simulink model "ASM_Traffic_new"  (R2024a)
settings: Solver=ode1  StartTime=SIM.tstart.v  StopTime=SIM.tend.v  FixedStep=SIM.StepSize.v  RelTol=1e-3
PostLoadFcn:
  | if any(exist('dsrtsu_mdlpostloadfcn', 'file') ~= 0), dsrtsu_mdlpostloadfcn('Execute', bdroot); end
  | try, asm_mdl_postloadfcn(bdroot, 'UpdateModel', 3600); catch, disp(lasterr); end,
InitFcn:
  | , if any(exist('rtifpga_mdlclblib', 'file') ~= 0), rtifpga_mdlclblib('Init', bdroot); end,
  | , if any(exist('dsmpb_private', 'file') ~= 0), dsmpb_private('dsmpb_mdlclblib', 'Init', bdroot); end,
undefined symbols (not defined in the file): _to_, a0b2, ASM_BrakeHydraulics_DemoSystems, ASM_VehicleDynamics_DemoSystems, b98103fe8ad365046cd0, BrakeCircuit, CPT, Crankshaft, DiscIntNeverNeededParam, dsmsi, FinalDriveAssembly, MDL, ModeSignals, Pos_BrakePedal_Maneuver, rad, RefSignals, s_to_rpm, SIM, SoftECU, Suspension, Tire, Transmission
libraries: ASM_Traffic_lib x135, simulink x100, ASM_Utils_lib x77, ASM_VehicleDynamics_lib x70, ASM_Environment_lib x22, dsmpblib x20, dsmsilib x15, MDLD_Utils_lib x10, ASM_BrakeHydraulics_lib x3
(part 23 of 63)

== system ASM_Traffic_new/Environment/GroundTruth/PlantModel/HostVehicle_Data_Access ==
  OSI_HV_Data : Inport
  Enable_HostVehicle_Data_Access[0Off|1On] : Constant
  HostVehicle_Data_Access : Subsystem
  Terminator{,1..23} (24 alike) : Terminator
  wires:
  HostVehicle_Data_Access/5(HV_Position_BB[x;y;z][m]) -> Terminator4/1
  HostVehicle_Data_Access/6(HV_Velocity_BB[x;y;z][m|s]) -> Terminator5/1
  HostVehicle_Data_Access/3(HV_ID[]) -> Terminator2/1
  HostVehicle_Data_Access/4(HV_Pos_BrakePedal[0_1]) -> Terminator3/1
  HostVehicle_Data_Access/2(Time_Stamp_Nanos[ns]) -> Terminator1/1
  Enable_HostVehicle_Data_Access[0Off|1On]/1 -> HostVehicle_Data_Access/1(Enable[0Off|1On])
  OSI_HV_Data/1 -> HostVehicle_Data_Access/2(OSI_HV_Data)
  HostVehicle_Data_Access/1(Time_Stamp_Seconds[s]) -> Terminator/1
  HostVehicle_Data_Access/7(HV_Acceleration_BB[x;y;z][m|s2]) -> Terminator6/1
  HostVehicle_Data_Access/8(HV_Orientation_BB[x;y;z][rad]) -> Terminator7/1
  HostVehicle_Data_Access/9(HV_Current_Curvature[1|m]) -> Terminator8/1
  HostVehicle_Data_Access/10(HV_Steering_Angle[rad]) -> Terminator9/1
  HostVehicle_Data_Access/11(HV_Steering_Angle_dt[rad|s]) -> Terminator10/1
  HostVehicle_Data_Access/12(HV_Steering_Torque[Nm]) -> Terminator11/1
  HostVehicle_Data_Access/13(HV_Pos_AccPedal[0_1]) -> Terminator12/1
  HostVehicle_Data_Access/14(HV_Pos_ClutchPedal[0_1]) -> Terminator13/1
  HostVehicle_Data_Access/15(HV_Gear[]) -> Terminator14/1
  HostVehicle_Data_Access/16(HV_Type_Engine[]) -> Terminator15/1
  HostVehicle_Data_Access/17(HV_n_Engine[rpm]) -> Terminator16/1
  HostVehicle_Data_Access/18(HV_Trq_Engine[Nm]) -> Terminator17/1
  HostVehicle_Data_Access/19(HV_Vehicle_Weight[kg]) -> Terminator18/1
  HostVehicle_Data_Access/20(HV_Vehicle_Operating_State[]) -> Terminator19/1
  HostVehicle_Data_Access/21(HV_WheelData_Axle_Idx[]) -> Terminator20/1
  HostVehicle_Data_Access/22(HV_WheelData_Wheel_Idx[]) -> Terminator21/1
  HostVehicle_Data_Access/23(HV_WheelData_Wheel_Speed[rad|s]) -> Terminator22/1
  HostVehicle_Data_Access/24(HV_WheelData_Wheel_Slip[]) -> Terminator23/1

== system ASM_Traffic_new/Environment/GroundTruth/PlantModel/ObjectDataStreams ==
  In : Inport
  Bus Selector14 : BusSelector  OutputSignals=DataStream_1[].DataStream_1[],DataStream_2[].DataStream_2[],DataStream_3[].DataStream_3[],DataStream_4[].DataStream_4[],DataStream_5[].DataStream_5[],DataStream_6[].DataStream_6[],DataStream_7[].DataStream_7[],DataStream_8[].DataStream_8[]
  Mux : Mux  Inputs=8
  Objects_DataStreams[] : Outport  VectorParamsAs1DForOutWhenUnconnected=off
  wires:
  Mux/1 -> Objects_DataStreams[]/1
  Bus Selector14/7 -> Mux/7  "<DataStream_7[]>"
  Bus Selector14/8 -> Mux/8  "<DataStream_8[]>"
  Bus Selector14/3 -> Mux/3  "<DataStream_3[]>"
  Bus Selector14/6 -> Mux/6  "<DataStream_6[]>"
  Bus Selector14/4 -> Mux/4  "<DataStream_4[]>"
  Bus Selector14/1 -> Mux/1  "<DataStream_1[]>"
  Bus Selector14/5 -> Mux/5  "<DataStream_5[]>"
  In/1 -> Bus Selector14/1
  Bus Selector14/2 -> Mux/2  "<DataStream_2[]>"

== system ASM_Traffic_new/Environment/GroundTruth/PlantModel/Running_Maneuver ==
  ManeuverState[] : Inport
  Brake : RelationalOperator  Operator===  OutDataTypeStr=boolean  InputSameDT=off
  Constant : Constant  Value=3
  Constant1 : Constant  Value=4
  Data Type Conversion : DataTypeConversion  OutDataTypeStr=double  SaturateOnIntegerOverflow=off  RndMeth=Floor
  Logical Operator : Logic  Operator=OR  AllPortsSameDT=off  OutDataTypeStr=boolean
  Run : RelationalOperator  Operator===  OutDataTypeStr=boolean  InputSameDT=off
  EnableRun[0Off|1On] : Outport  VectorParamsAs1DForOutWhenUnconnected=off
  wires:
  Run/1 -> Logical Operator/1
  ManeuverState[]/1 -> Brake/1, Run/1
  Constant1/1 -> Brake/2
  Logical Operator/1 -> Data Type Conversion/1
  Constant/1 -> Run/2
  Brake/1 -> Logical Operator/2
  Data Type Conversion/1 -> EnableRun[0Off|1On]/1

== system ASM_Traffic_new/Environment/GroundTruth/PlantModel/TrafficLight_Counter ==
  In : Inport
  Bus Selector14 : BusSelector  OutputSignals=TrafficLight_Counter_1[].TrafficLight_Counter_1[],TrafficLight_Counter_2.TrafficLight_Counter_2[],TrafficLight_Counter_3.TrafficLight_Counter_3[],TrafficLight_Counter_4[].TrafficLight_Counter_4[]
  Mux2 : Mux
  TrafficLight_Counter[] : Outport  VectorParamsAs1DForOutWhenUnconnected=off
  wires:
  Bus Selector14/1 -> Mux2/1  "<TrafficLight_Counter_1[]>"
  In/1 -> Bus Selector14/1
  Bus Selector14/3 -> Mux2/3  "<TrafficLight_Counter_3[]>"
  Bus Selector14/2 -> Mux2/2  "<TrafficLight_Counter_2[]>"
  Bus Selector14/4 -> Mux2/4  "<TrafficLight_Counter_4[]>"
  Mux2/1 -> TrafficLight_Counter[]/1

== system ASM_Traffic_new/Environment/GroundTruth/PlantModel/VehicleBasics ==
  In : Inport
  OSIGroundTruth : Inport  Port=2
  Bus Selector : BusSelector  OutputSignals=Interface_In.ExternalModel.m_TotalVehicle[kg],Interface_In.ExternalModel.State_StartButton[-2|-1|0|1|2|3]
  Bus Selector1 : BusSelector  OutputSignals=HostVehicle_Data_VehicleBasics[].Mode_OperatingState[1Stim|2Int],HostVehicle_Data_VehicleBasics[].Stim_OperatingState[]
  Multiport Switch : MultiPortSwitch  Inputs=2  SaturateOnIntegerOverflow=off  InputSameDT=off
  StartButton_Mapping : Subsystem
  m_TotalVehicle[kg] : Outport  VectorParamsAs1DForOutWhenUnconnected=off
  OperatingState[] : Outport  Port=2  VectorParamsAs1DForOutWhenUnconnected=off
  wires:
  Multiport Switch/1 -> OperatingState[]/1  "OperatingState[]"
  Bus Selector1/2 -> Multiport Switch/2  "<Stim_OperatingState[]>"
  Bus Selector1/1 -> Multiport Switch/1  "<Mode_OperatingState[1Stim|2Int]>"
  OSIGroundTruth/1 -> Bus Selector1/1
  In/1 -> Bus Selector/1
  Bus Selector/1 -> m_TotalVehicle[kg]/1  "<m_TotalVehicle[kg]>"
  Bus Selector/2 -> StartButton_Mapping/1(State_StartButton[-2|-1|0|1|2|3])  "<State_StartButton[-2|-1|0|1|2|3]>"
  StartButton_Mapping/1(OperatingState[]) -> Multiport Switch/3

== system ASM_Traffic_new/Environment/GroundTruth/PlantModel/VehicleBrakeSystem ==
  In : Inport
  Bus Selector25 : BusSelector  OutputSignals=Interface_In.ExternalModel.Pos_BrakePedal[%]
  Gain : Gain  Gain=1/100
  Pos_BrakePedal[0_1] : Outport
  wires:
  Bus Selector25/1 -> Gain/1  "<Pos_BrakePedal[%]>"
  In/1 -> Bus Selector25/1
  Gain/1 -> Pos_BrakePedal[0_1]/1

== system ASM_Traffic_new/Environment/GroundTruth/PlantModel/VehicleLocalization ==
  In : Inport
  Bus Selector : BusSelector  OutputSignals=Longitude[deg],Latitude[deg]
  Bus Selector10 : BusSelector  OutputSignals=Maneuver.Plant.ManeuverScheduler.Parameters.Object_Type_ID[]
  Bus Selector2 : BusSelector  OutputSignals=Interface_In.ExternalModel.Pos_Vehicle_CoorSys_E[x;y;z][m]
  Bus Selector22 : BusSelector  OutputSignals=Road.Plant.UserSignals_Customized
  Bus Selector3 : BusSelector  OutputSignals=Object_Properties_Box.PosVec_x_CenterPnt_Object[m],Object_Properties_Box.PosVec_y_CenterPnt_Object[m],Object_Properties_Box.PosVec_z_CenterPnt_Object[m]
  Bus Selector4 : BusSelector  OutputSignals=Interface_In.ExternalModel.Angle_Vehicle_CoorSys_E[x;y;z][deg]
  Bus Selector5 : BusSelector  OutputSignals=Traffic.Plant.ObjectParameters.TrafficObjects.TrafficObject_Type_Data[]
  COORDINATE_TRANSFORMATION_B_TO_A : ASM_Utils_lib/MatrixOperations/COORDINATE_TRANSFORMATION_B_TO_A  ASMLibrary2Check=ASM_Traffic_lib
  ChangeLabel : Subsystem
      mask Display: disp('')
  Demux : Demux  Outputs=3
  Demux1 : Demux  Outputs=3
  GPS_POSITION : ASM_Environment_lib/Environment/Road/GPS_POSITION  Tag=ASM_SUBCOMPONENT  ASMProperties=struct('Name','GPS_POSITION','Version','3.0','Library','ASM_Environment_lib')  ASMInstanceName=GPS_Position  ASMInstanceID=2
      settings: AttributesFormatString=Instance Name: %<ASMInstanceName>\nInstance ID: %<ASMInstanceID>
  Mux : Mux  Inputs=3
  OBJECT_PROPERTIES_BOX : ASM_Traffic_lib/Objects/OBJECT_PROPERTIES_BOX  ASMProperties=struct('Name','OBJECT_PROPERTIES_BOX','Version','2.0','Library','ASM_Traffic_lib')  ASMInstanceName=object_properties_box  ASMInstanceID=1
  Terminator : Terminator
  Terminator1 : Terminator
  Pos_Veh_BoundingBox_GPS[Long;Lat;Alt][deg;deg;m] : Outport
  wires:
  Bus Selector22/1 -> GPS_POSITION/1  "<UserSignals_Customized>"
  GPS_POSITION/1 -> Terminator/1
  GPS_POSITION/2 -> Bus Selector/1
  Bus Selector/1 -> Mux/1  "<Longitude[deg]>"
  Bus Selector/2 -> Mux/2  "<Latitude[deg]>"
  Mux/1 -> Pos_Veh_BoundingBox_GPS[Long;Lat;Alt][deg;deg;m]/1
  Bus Selector10/1 -> OBJECT_PROPERTIES_BOX/1  "<Object_Type_ID[]>"
  In/1 -> Bus Selector4/1, Bus Selector5/1, Bus Selector10/1, Bus Selector2/1, Bus Selector22/1
  Bus Selector5/1 -> OBJECT_PROPERTIES_BOX/2  "<TrafficObject_Type_Data[]>"
  OBJECT_PROPERTIES_BOX/1 -> Terminator1/1
  Bus Selector2/1 -> Demux/1  "<Pos_Vehicle_CoorSys_E[x;y;z][m]>"
  Demux/1 -> COORDINATE_TRANSFORMATION_B_TO_A/1
  Demux/2 -> COORDINATE_TRANSFORMATION_B_TO_A/2
  Demux/3 -> COORDINATE_TRANSFORMATION_B_TO_A/3
  Bus Selector3/2 -> COORDINATE_TRANSFORMATION_B_TO_A/5  "<PosVec_y_CenterPnt_Object[m]>"
  Bus Selector3/1 -> COORDINATE_TRANSFORMATION_B_TO_A/4  "<PosVec_x_CenterPnt_Object[m]>"
  Bus Selector3/3 -> COORDINATE_TRANSFORMATION_B_TO_A/6  "<PosVec_z_CenterPnt_Object[m]>"
  OBJECT_PROPERTIES_BOX/2 -> Bus Selector3/1
  Demux1/1 -> COORDINATE_TRANSFORMATION_B_TO_A/7
  Demux1/2 -> COORDINATE_TRANSFORMATION_B_TO_A/8
  Demux1/3 -> COORDINATE_TRANSFORMATION_B_TO_A/9
  COORDINATE_TRANSFORMATION_B_TO_A/3 -> ChangeLabel/1(In1)  "Pos_z_CoorSysE[m]"
  COORDINATE_TRANSFORMATION_B_TO_A/1 -> GPS_POSITION/2  "Pos_x_CoorSysE[m]"
  COORDINATE_TRANSFORMATION_B_TO_A/2 -> GPS_POSITION/3  "Pos_y_CoorSysE[m]"
  Bus Selector4/1 -> Demux1/1  "<Angle_Vehicle_CoorSys_E[x;y;z][deg]>"
  ChangeLabel/1(Out1) -> Mux/3  "Altitude[m]"

== system ASM_Traffic_new/Environment/GroundTruth/PlantModel/VehiclePowertrain ==
  In : Inport
  Bus Selector : BusSelector  OutputSignals=Interface_In.ExternalModel.Pos_AccPedal[%],Interface_In.ExternalModel.Pos_ClutchPedal[%],Interface_In.ExternalModel.Gear[],Interface_In.ExternalModel.n_Engine_1[rpm],Interface_In.ExternalModel.n_Engine_2[rpm],Interface_In.ExternalModel.Type_Engine_1[0Unkown|1Other|2Otto|3Diesel|4Electric],Interface_In.ExternalModel.Type_Engine_2[0Unkown|1Other|2Otto|3Diesel|4Electric],Interface_In.ExternalModel.Trq_Engine_1[Nm],Interface_In.ExternalModel.Trq_Engine_2[Nm]
  Gain : Gain  Gain=1/100
  Gain1 : Gain  Gain=1/100
  Mux : Mux  Inputs=2
  Mux1 : Mux  Inputs=2
  Mux2 : Mux  Inputs=2
  Pos_AccPedal[0_1] : Outport  VectorParamsAs1DForOutWhenUnconnected=off
  Pos_ClutchPedal[0_1] : Outport  Port=2  VectorParamsAs1DForOutWhenUnconnected=off
  Gear[] : Outport  Port=3  VectorParamsAs1DForOutWhenUnconnected=off
  n_Engine[rpm] : Outport  Port=4  VectorParamsAs1DForOutWhenUnconnected=off
  Type_Engine[0Unkown|1Other|2Otto|3Diesel|4Electric] : Outport  Port=5  VectorParamsAs1DForOutWhenUnconnected=off
  Trq_Engine[Nm] : Outport  Port=6  VectorParamsAs1DForOutWhenUnconnected=off
  wires:
  Bus Selector/3 -> Gear[]/1  "<Gear[]>"
  Bus Selector/4 -> Mux/1  "<n_Engine_1[rpm]>"
  Bus Selector/2 -> Gain1/1  "<Pos_ClutchPedal[%]>"
  In/1 -> Bus Selector/1
  Bus Selector/1 -> Gain/1  "<Pos_AccPedal[%]>"
  Mux/1 -> n_Engine[rpm]/1
  Bus Selector/5 -> Mux/2  "<n_Engine_2[rpm]>"
  Bus Selector/6 -> Mux1/1  "<Type_Engine_1[0Unkown|1Other|2Otto|3Diesel|4Electric]>"
  Bus Selector/7 -> Mux1/2  "<Type_Engine_2[0Unkown|1Other|2Otto|3Diesel|4Electric]>"
  Bus Selector/8 -> Mux2/1  "<Trq_Engine_1[Nm]>"
  Bus Selector/9 -> Mux2/2  "<Trq_Engine_2[Nm]>"
  Mux1/1 -> Type_Engine[0Unkown|1Other|2Otto|3Diesel|4Electric]/1
  Mux2/1 -> Trq_Engine[Nm]/1
  Gain/1 -> Pos_AccPedal[0_1]/1
  Gain1/1 -> Pos_ClutchPedal[0_1]/1

== system ASM_Traffic_new/Environment/GroundTruth/PlantModel/VehicleSteering ==
  In : Inport
  Bus Selector24 : BusSelector  OutputSignals=Interface_In.ExternalModel.Angle_SteeringWheel_SteeringSystem[deg],Interface_In.ExternalModel.Angle_SteeringWheel_dt_SteeringSystem[deg|s],Interface_In.ExternalModel.Trq_SteeringWheel_SteeringSystem[Nm]
  UnitConversion : ASM_Utils_lib/UnitConversion/UnitConversion  Selection=deg_to_rad
  UnitConversion1 : ASM_Utils_lib/UnitConversion/UnitConversion  Selection=deg_to_rad
  Angle_SteeringWheel_SteeringSystem[rad] : Outport  VectorParamsAs1DForOutWhenUnconnected=off
  Angle_SteeringWheel_dt_SteeringSystem[rad|s] : Outport  Port=2  VectorParamsAs1DForOutWhenUnconnected=off
  Trq_SteeringWheel_SteeringSystem[Nm] : Outport  Port=3  VectorParamsAs1DForOutWhenUnconnected=off
  wires:
  In/1 -> Bus Selector24/1
  Bus Selector24/1 -> UnitConversion/1  "<Angle_SteeringWheel_SteeringSystem[deg]>"
  Bus Selector24/2 -> UnitConversion1/1  "<Angle_SteeringWheel_dt_SteeringSystem[deg|s]>"
  Bus Selector24/3 -> Trq_SteeringWheel_SteeringSystem[Nm]/1  "<Trq_SteeringWheel_SteeringSystem[Nm]>"
  UnitConversion/1 -> Angle_SteeringWheel_SteeringSystem[rad]/1
  UnitConversion1/1 -> Angle_SteeringWheel_dt_SteeringSystem[rad|s]/1

== system ASM_Traffic_new/Environment/GroundTruth/PlantModel/VehicleWheels ==
  In : Inport
  OSIGroundTruth : Inport  Port=2
  Bus Selector1 : BusSelector  OutputSignals=HostVehicle_Data_VehicleWheels[].Axle_Idx[],HostVehicle_Data_VehicleWheels[].Wheel_Idx[]
  Bus Selector37 : BusSelector  OutputSignals=Interface_In.ExternalModel.omega_Wheel[rad|s],Interface_In.ExternalModel.Slip_x_Wheel[]
  Axle_Idx[] : Outport  VectorParamsAs1DForOutWhenUnconnected=off
  Wheel_Idx[] : Outport  Port=2  VectorParamsAs1DForOutWhenUnconnected=off
  omega_Wheel[rad|s] : Outport  Port=3  VectorParamsAs1DForOutWhenUnconnected=off
  Slip_x_Wheel[] : Outport  Port=4  VectorParamsAs1DForOutWhenUnconnected=off
  wires:
  In/1 -> Bus Selector37/1
  Bus Selector37/1 -> omega_Wheel[rad|s]/1  "<omega_Wheel[rad|s]>"
  Bus Selector37/2 -> Slip_x_Wheel[]/1  "<Slip_x_Wheel[]>"
  Bus Selector1/1 -> Axle_Idx[]/1  "<Axle_Idx[]>"
  Bus Selector1/2 -> Wheel_Idx[]/1  "<Wheel_Idx[]>"
  OSIGroundTruth/1 -> Bus Selector1/1

== system ASM_Traffic_new/Environment/GroundTruth/UserInterface/ASMSignalBus_Plant ==
  In : Inport
  Terminator_1 : Terminator
  tag scope: ASMBUS_Traffic_GroundTruth=global
  wires:
  In/1 -> [ASMBUS_Traffic_GroundTruth]
  [ASMBUS_Traffic_GroundTruth] -> Terminator_1/1

== system ASM_Traffic_new/Environment/GroundTruth/UserInterface/DISP_Plant ==
  In : Inport
  Bus Selector : BusSelector  OutputSignals=Control.Interface_Mode[0Off|1ObjOnly|2ObjAndLanes]
  Bus Selector1 : BusSelector  OutputSignals=Data_Access.Num_MovObj[],Data_Access.Num_MovObj_in_GT_Area[],Data_Access.Num_StatObj[],Data_Access.Num_StatObj_in_GT_Area[],Data_Access.Num_Laneboundaries[],Data_Access.Num_Lanes[],Data_Access.Num_TrfLights[],Data_Access.Num_TrfLights_in_GT_Area[],Data_Access.Num_TrfSigns[],Data_Access.Num_TrfSigns_in_GT_Area[]
  Bus Selector2 : BusSelector  OutputSignals=Data_Access.Num_MovObj[],Data_Access.Num_MovObj_in_GT_Area[],Data_Access.Num_StatObj[],Data_Access.Num_StatObj_in_GT_Area[],Data_Access.Num_Laneboundaries[],Data_Access.Num_Lanes[],Data_Access.Num_TrfLights[],Data_Access.Num_TrfLights_in_GT_Area[],Data_Access.Num_TrfSigns[],Data_Access.Num_TrfSigns_in_GT_Area[]
  Interface_Mode : Scope
  Interface_Mode[0Off|1ObjOnly|2ObjAndLanes] : Subsystem
      mask Display: disp('')
  Interface_Mode_Disp : Display
  Lanes_Laneboundaries : Scope  NumInputPorts=2
  MovObj : Scope  NumInputPorts=2
  Num_Laneboundaries : Display
  Num_Laneboundaries[] : Subsystem
      mask Display: disp('')
  Num_Lanes : Display
  Num_Lanes[] : Subsystem
      mask Display: disp('')
  Num_MovObj : Display
  Num_MovObj[] : Subsystem
      mask Display: disp('')
  Num_MovObj_in_GT_Area : Display
  Num_MovObj_in_GT_Area[] : Subsystem
      mask Display: disp('')
  Num_StatObj : Display
  Num_StatObj[] : Subsystem
      mask Display: disp('')
  Num_StatObj_in_GT_Area : Display
  Num_StatObj_in_GT_Area[] : Subsystem
      mask Display: disp('')
  Num_TrfLights : Display
  Num_TrfLights[] : Subsystem
      mask Display: disp('')
  Num_TrfLights_in_GT_Area : Display
  Num_TrfLights_in_GT_Area[] : Subsystem
      mask Display: disp('')
  Num_TrfSigns : Display
  Num_TrfSigns[] : Subsystem
      mask Display: disp('')
  Num_TrfSigns_in_GT_Area : Display
  Num_TrfSigns_in_GT_Area[] : Subsystem
      mask Display: disp('')
  StatObj : Scope  NumInputPorts=2
  TrfLights : Scope  NumInputPorts=2
  TrfSigns : Scope  NumInputPorts=2
  wires:
  In/1 -> Bus Selector2/1, Bus Selector1/1, Bus Selector/1
  Bus Selector/1 -> Interface_Mode[0Off|1ObjOnly|2ObjAndLanes]/1(In1)  "<Interface_Mode[0Off|1ObjOnly|2ObjAndLanes]>"
  Bus Selector1/1 -> Num_MovObj[]/1(In1)  "<Num_MovObj[]>"
  Bus Selector1/2 -> Num_MovObj_in_GT_Area[]/1(In1)  "<Num_MovObj_in_GT_Area[]>"
  Bus Selector1/3 -> Num_StatObj[]/1(In1)  "<Num_StatObj[]>"
  Bus Selector1/4 -> Num_StatObj_in_GT_Area[]/1(In1)  "<Num_StatObj_in_GT_Area[]>"
  Bus Selector1/5 -> Num_Laneboundaries[]/1(In1)  "<Num_Laneboundaries[]>"
  Bus Selector1/6 -> Num_Lanes[]/1(In1)  "<Num_Lanes[]>"
  Bus Selector1/7 -> Num_TrfLights[]/1(In1)  "<Num_TrfLights[]>"
  Bus Selector1/8 -> Num_TrfLights_in_GT_Area[]/1(In1)  "<Num_TrfLights_in_GT_Area[]>"
  Bus Selector1/9 -> Num_TrfSigns[]/1(In1)  "<Num_TrfSigns[]>"
  Bus Selector1/10 -> Num_TrfSigns_in_GT_Area[]/1(In1)  "<Num_TrfSigns_in_GT_Area[]>"
  Num_MovObj[]/1(Out1) -> MovObj/1  "Num_MovObj[]"
  Num_MovObj_in_GT_Area[]/1(Out1) -> MovObj/2  "Num_MovObj_in_GT_Area[]"
  Interface_Mode[0Off|1ObjOnly|2ObjAndLanes]/1(Out1) -> Interface_Mode_Disp/1, Interface_Mode/1  "Interface_Mode[0Off|1ObjOnly|2ObjAndLanes]"
  Num_StatObj[]/1(Out1) -> StatObj/1  "Num_StatObj[]"
  Num_StatObj_in_GT_Area[]/1(Out1) -> StatObj/2  "Num_StatObj_in_GT_Area[]"
  Num_Laneboundaries[]/1(Out1) -> Lanes_Laneboundaries/1  "Num_Laneboundaries[]"
  Num_Lanes[]/1(Out1) -> Lanes_Laneboundaries/2  "Num_Lanes[]"
  Num_TrfLights[]/1(Out1) -> TrfLights/1  "Num_TrfLights[]"
  Num_TrfLights_in_GT_Area[]/1(Out1) -> TrfLights/2  "Num_TrfLights_in_GT_Area[]"
  Num_TrfSigns[]/1(Out1) -> TrfSigns/1  "Num_TrfSigns[]"
  Num_TrfSigns_in_GT_Area[]/1(Out1) -> TrfSigns/2  "Num_TrfSigns_in_GT_Area[]"
  Bus Selector2/1 -> Num_MovObj/1  "<Num_MovObj[]>"
  Bus Selector2/2 -> Num_MovObj_in_GT_Area/1  "<Num_MovObj_in_GT_Area[]>"
  Bus Selector2/3 -> Num_StatObj/1  "<Num_StatObj[]>"
  Bus Selector2/4 -> Num_StatObj_in_GT_Area/1  "<Num_StatObj_in_GT_Area[]>"
  Bus Selector2/5 -> Num_Laneboundaries/1  "<Num_Laneboundaries[]>"
  Bus Selector2/6 -> Num_Lanes/1  "<Num_Lanes[]>"
  Bus Selector2/7 -> Num_TrfLights/1  "<Num_TrfLights[]>"
  Bus Selector2/8 -> Num_TrfLights_in_GT_Area/1  "<Num_TrfLights_in_GT_Area[]>"
  Bus Selector2/9 -> Num_TrfSigns/1  "<Num_TrfSigns[]>"
  Bus Selector2/10 -> Num_TrfSigns_in_GT_Area/1  "<Num_TrfSigns_in_GT_Area[]>"

== system ASM_Traffic_new/Environment/GroundTruth/UserInterface/PAR_Plant ==
  Interface_In : Inport
  In : Inport  Port=2
  Bus Creator : BusCreator  Inputs=1
  Bus Creator1 : BusCreator  Inputs=9
  Country_Code[] : Constant  Tag=AD:ASM_Sw_SpeedLimit_Source[1Manual|2RoadScenery]
  Ego_Vehicle : Subsystem
  Enable_HostVehicle_Data[0Off|1On] : Constant  Tag=AD:ASM_Sw_SpeedLimit_Source[1Manual|2RoadScenery]
  Environmental_Conditions : Subsystem
  Fellow_Vehicles : Subsystem
  HostVehicle_Data_AutomatedDrivingFunction : Subsystem
  HostVehicle_Data_VehicleBasics : Subsystem
  HostVehicle_Data_VehicleWheels : Subsystem
  Terminator1 : Terminator
  TrafficLight_Counter : Subsystem
  Out : Outport  VectorParamsAs1DForOutWhenUnconnected=off
  wires:
  In/1 -> Terminator1/1
  Bus Creator/1 -> Out/1  "UserInterface"
  Bus Creator1/1 -> Bus Creator/1  "OSIGroundTruth"
  Enable_HostVehicle_Data[0Off|1On]/1 -> Bus Creator1/6  "Enable_HostVehicle_Data[0Off|1On]"
  HostVehicle_Data_VehicleWheels/1(HostVehicle_Data_VehicleWheels[]) -> Bus Creator1/7
  Ego_Vehicle/1(Ego_Vehicle[]) -> Bus Creator1/2
  Country_Code[]/1 -> Bus Creator1/1  "Country_Code[]"
  Fellow_Vehicles/1(Fellow_Vehicles[]) -> Bus Creator1/3
  Interface_In/1 -> HostVehicle_Data_AutomatedDrivingFunction/1(Interface_In), Fellow_Vehicles/1(Interface_In), Ego_Vehicle/1(Interface_In)
  Environmental_Conditions/1(Environmental_Conditions[]) -> Bus Creator1/4
  TrafficLight_Counter/1(TrafficLight_Counter[]) -> Bus Creator1/5
  HostVehicle_Data_AutomatedDrivingFunction/1(HostVehicle_Data_AutomatedDrivingFunction[]) -> Bus Creator1/9
  HostVehicle_Data_VehicleBasics/1(HostVehicle_Data_VehicleBasics[]) -> Bus Creator1/8

== system ASM_Traffic_new/Environment/Interface_In/ModelSignals/ACC_State[1OFF|2Standby|3ON]_ ==
  In1 : Inport
  DummyGain : Gain  SaturateOnIntegerOverflow=on  OutDataTypeStr=Inherit: Same as input  ParamDataTypeStr=Inherit: Same as input
  Out1 : Outport  VectorParamsAs1DForOutWhenUnconnected=off
  wires:
  DummyGain/1 -> Out1/1
  In1/1 -> DummyGain/1

== system ASM_Traffic_new/Environment/Interface_In/ModelSignals/AEB[0|1]_ ==
  In1 : Inport
  Gain : Gain  SaturateOnIntegerOverflow=on  OutDataTypeStr=Inherit: Same as input  ParamDataTypeStr=Inherit: Same as input
  Out1 : Outport  VectorParamsAs1DForOutWhenUnconnected=off
  wires:
  Gain/1 -> Out1/1
  In1/1 -> Gain/1

== system ASM_Traffic_new/Environment/Interface_In/ModelSignals/Active_CP_VehDyn_Trailer[]_ ==
  In1 : Inport
  Gain : Gain  SaturateOnIntegerOverflow=on  OutDataTypeStr=Inherit: Same as input  ParamDataTypeStr=Inherit: Same as input
  Out1 : Outport  VectorParamsAs1DForOutWhenUnconnected=off
  wires:
  In1/1 -> Gain/1
  Gain/1 -> Out1/1

== system ASM_Traffic_new/Environment/Interface_In/ModelSignals/Angle_SteeringWheel[deg]_ ==
  In1 : Inport
  DummyGain : Gain  SaturateOnIntegerOverflow=on  OutDataTypeStr=Inherit: Same as input  ParamDataTypeStr=Inherit: Same as input
  Out1 : Outport  VectorParamsAs1DForOutWhenUnconnected=off
  wires:
  DummyGain/1 -> Out1/1
  In1/1 -> DummyGain/1

== system ASM_Traffic_new/Environment/Interface_In/ModelSignals/Angle_SteeringWheel_SteeringSystem[deg]_ ==
  In1 : Inport
  Gain : Gain  SaturateOnIntegerOverflow=on  OutDataTypeStr=Inherit: Same as input  ParamDataTypeStr=Inherit: Same as input
  Out1 : Outport  VectorParamsAs1DForOutWhenUnconnected=off
  wires:
  Gain/1 -> Out1/1
  In1/1 -> Gain/1

== system ASM_Traffic_new/Environment/Interface_In/ModelSignals/Angle_SteeringWheel_dt_SteeringSystem[deg|s]_ ==
  In1 : Inport
  Gain : Gain  SaturateOnIntegerOverflow=on  OutDataTypeStr=Inherit: Same as input  ParamDataTypeStr=Inherit: Same as input
  Out1 : Outport  VectorParamsAs1DForOutWhenUnconnected=off
  wires:
  Gain/1 -> Out1/1
  In1/1 -> Gain/1

== system ASM_Traffic_new/Environment/Interface_In/ModelSignals/Angle_Vehicle_CoorSys_E[x;y;z][deg]_ ==
  In1 : Inport
  Gain : Gain  SaturateOnIntegerOverflow=on  OutDataTypeStr=Inherit: Same as input  ParamDataTypeStr=Inherit: Same as input
  Out1 : Outport  VectorParamsAs1DForOutWhenUnconnected=off
  wires:
  Gain/1 -> Out1/1
  In1/1 -> Gain/1

== system ASM_Traffic_new/Environment/Interface_In/ModelSignals/Coef_RollingRes[FL;FR;RL;RR][]_ ==
  In1 : Inport
  Gain : Gain  SaturateOnIntegerOverflow=on  OutDataTypeStr=Inherit: Same as input  ParamDataTypeStr=Inherit: Same as input
  Out1 : Outport  VectorParamsAs1DForOutWhenUnconnected=off
  wires:
  Gain/1 -> Out1/1
  In1/1 -> Gain/1

== system ASM_Traffic_new/Environment/Interface_In/ModelSignals/Coef_RollingRes_Mean[]_ ==
  In1 : Inport
  Gain : Gain  SaturateOnIntegerOverflow=on  OutDataTypeStr=Inherit: Same as input  ParamDataTypeStr=Inherit: Same as input
  Out1 : Outport  VectorParamsAs1DForOutWhenUnconnected=off
  wires:
  In1/1 -> Gain/1
  Gain/1 -> Out1/1

== system ASM_Traffic_new/Environment/Interface_In/ModelSignals/Const_r_unloaded_Tire_Mean[m]_ ==
  In1 : Inport
  Gain : Gain  SaturateOnIntegerOverflow=on  OutDataTypeStr=Inherit: Same as input  ParamDataTypeStr=Inherit: Same as input
  Out1 : Outport  VectorParamsAs1DForOutWhenUnconnected=off
  wires:
  In1/1 -> Gain/1
  Gain/1 -> Out1/1

== system ASM_Traffic_new/Environment/Interface_In/ModelSignals/CorneringStiffness[FL;FR;RL;RR][N]_ ==
  In1 : Inport
  Gain : Gain  SaturateOnIntegerOverflow=on  OutDataTypeStr=Inherit: Same as input  ParamDataTypeStr=Inherit: Same as input
  Out1 : Outport  VectorParamsAs1DForOutWhenUnconnected=off
  wires:
  Gain/1 -> Out1/1
  In1/1 -> Gain/1

== system ASM_Traffic_new/Environment/Interface_In/ModelSignals/Driver_Override_ACC_Active[0Off|1On]_ ==
  In1 : Inport
  DummyGain : Gain  SaturateOnIntegerOverflow=on  OutDataTypeStr=Inherit: Same as input  ParamDataTypeStr=Inherit: Same as input
  Out1 : Outport  VectorParamsAs1DForOutWhenUnconnected=off
  wires:
  DummyGain/1 -> Out1/1
  In1/1 -> DummyGain/1

== system ASM_Traffic_new/Environment/Interface_In/ModelSignals/Driver_Override_ACC_Reason[0NoOverride|1BrakePedal|2AccPedal]_ ==
  In1 : Inport
  DummyGain : Gain  SaturateOnIntegerOverflow=on  OutDataTypeStr=Inherit: Same as input  ParamDataTypeStr=Inherit: Same as input
  Out1 : Outport  VectorParamsAs1DForOutWhenUnconnected=off
  wires:
  DummyGain/1 -> Out1/1
  In1/1 -> DummyGain/1

== system ASM_Traffic_new/Environment/Interface_In/ModelSignals/FCW[0|1]_ ==
  In1 : Inport
  Gain : Gain  SaturateOnIntegerOverflow=on  OutDataTypeStr=Inherit: Same as input  ParamDataTypeStr=Inherit: Same as input
  Out1 : Outport  VectorParamsAs1DForOutWhenUnconnected=off
  wires:
  Gain/1 -> Out1/1
  In1/1 -> Gain/1

== system ASM_Traffic_new/Environment/Interface_In/ModelSignals/Gear[]_ ==
  In1 : Inport
  DummyGain : Gain  SaturateOnIntegerOverflow=on  OutDataTypeStr=Inherit: Same as input  ParamDataTypeStr=Inherit: Same as input
  Out1 : Outport  VectorParamsAs1DForOutWhenUnconnected=off
  wires:
  In1/1 -> DummyGain/1
  DummyGain/1 -> Out1/1

== system ASM_Traffic_new/Environment/Interface_In/ModelSignals/Mode_Drivetrain[1|2|3|4|5]_ ==
  In1 : Inport
  Gain : Gain  SaturateOnIntegerOverflow=on  OutDataTypeStr=Inherit: Same as input  ParamDataTypeStr=Inherit: Same as input
  Out1 : Outport  VectorParamsAs1DForOutWhenUnconnected=off
  wires:
  In1/1 -> Gain/1
  Gain/1 -> Out1/1

== system ASM_Traffic_new/Environment/Interface_In/ModelSignals/Mode_Transmission[1Manual|2Automatic]_ ==
  In1 : Inport
  Gain : Gain  SaturateOnIntegerOverflow=on  OutDataTypeStr=Inherit: Same as input  ParamDataTypeStr=Inherit: Same as input
  Out1 : Outport  VectorParamsAs1DForOutWhenUnconnected=off
  wires:
  In1/1 -> Gain/1
  Gain/1 -> Out1/1

== system ASM_Traffic_new/Environment/Interface_In/ModelSignals/Pos_AccPedal[%]_ ==
  In1 : Inport
  DummyGain : Gain  SaturateOnIntegerOverflow=on  OutDataTypeStr=Inherit: Same as input  ParamDataTypeStr=Inherit: Same as input
  Out1 : Outport  VectorParamsAs1DForOutWhenUnconnected=off
  wires:
  In1/1 -> DummyGain/1
  DummyGain/1 -> Out1/1

== system ASM_Traffic_new/Environment/Interface_In/ModelSignals/Pos_BrakePedal[%]_ ==
  In1 : Inport
  DummyGain : Gain  SaturateOnIntegerOverflow=on  OutDataTypeStr=Inherit: Same as input  ParamDataTypeStr=Inherit: Same as input
  Out1 : Outport  VectorParamsAs1DForOutWhenUnconnected=off
  wires:
  In1/1 -> DummyGain/1
  DummyGain/1 -> Out1/1

== system ASM_Traffic_new/Environment/Interface_In/ModelSignals/Pos_CP_FL2_Trailer_CoorSys_E[x;y][m]_ ==
  In1 : Inport
  Gain : Gain  SaturateOnIntegerOverflow=on  OutDataTypeStr=Inherit: Same as input  ParamDataTypeStr=Inherit: Same as input
  Out1 : Outport  VectorParamsAs1DForOutWhenUnconnected=off
  wires:
  Gain/1 -> Out1/1
  In1/1 -> Gain/1

== system ASM_Traffic_new/Environment/Interface_In/ModelSignals/Pos_CP_FL_CoorSys_E[x;y][m]_ ==
  In1 : Inport
  Gain : Gain  SaturateOnIntegerOverflow=on  OutDataTypeStr=Inherit: Same as input  ParamDataTypeStr=Inherit: Same as input
  Out1 : Outport  VectorParamsAs1DForOutWhenUnconnected=off
  wires:
  Gain/1 -> Out1/1
  In1/1 -> Gain/1

== system ASM_Traffic_new/Environment/Interface_In/ModelSignals/Pos_CP_FL_Trailer_CoorSys_E[x;y][m]_ ==
  In1 : Inport
  Gain : Gain  SaturateOnIntegerOverflow=on  OutDataTypeStr=Inherit: Same as input  ParamDataTypeStr=Inherit: Same as input
  Out1 : Outport  VectorParamsAs1DForOutWhenUnconnected=off
  wires:
  Gain/1 -> Out1/1
  In1/1 -> Gain/1

== system ASM_Traffic_new/Environment/Interface_In/ModelSignals/Pos_CP_FR2_Trailer_CoorSys_E[x;y][m]_ ==
  In1 : Inport
  Gain : Gain  SaturateOnIntegerOverflow=on  OutDataTypeStr=Inherit: Same as input  ParamDataTypeStr=Inherit: Same as input
  Out1 : Outport  VectorParamsAs1DForOutWhenUnconnected=off
  wires:
  Gain/1 -> Out1/1
  In1/1 -> Gain/1

== system ASM_Traffic_new/Environment/Interface_In/ModelSignals/Pos_CP_FR_CoorSys_E[x;y][m]_ ==
  In1 : Inport
  Gain : Gain  SaturateOnIntegerOverflow=on  OutDataTypeStr=Inherit: Same as input  ParamDataTypeStr=Inherit: Same as input
  Out1 : Outport  VectorParamsAs1DForOutWhenUnconnected=off
  wires:
  In1/1 -> Gain/1
  Gain/1 -> Out1/1

== system ASM_Traffic_new/Environment/Interface_In/ModelSignals/Pos_CP_FR_Trailer_CoorSys_E[x;y][m]_ ==
  In1 : Inport
  Gain : Gain  SaturateOnIntegerOverflow=on  OutDataTypeStr=Inherit: Same as input  ParamDataTypeStr=Inherit: Same as input
  Out1 : Outport  VectorParamsAs1DForOutWhenUnconnected=off
  wires:
  Gain/1 -> Out1/1
  In1/1 -> Gain/1

== system ASM_Traffic_new/Environment/Interface_In/ModelSignals/Pos_CP_Front_CoorSys_E[x;y][m]_ ==
  In1 : Inport
  Gain : Gain  SaturateOnIntegerOverflow=on  OutDataTypeStr=Inherit: Same as input  ParamDataTypeStr=Inherit: Same as input
  Out1 : Outport  VectorParamsAs1DForOutWhenUnconnected=off
  wires:
  In1/1 -> Gain/1
  Gain/1 -> Out1/1

== system ASM_Traffic_new/Environment/Interface_In/ModelSignals/Pos_CP_R2L2_CoorSys_E[x;y][m]_ ==
  In1 : Inport
  Gain : Gain  SaturateOnIntegerOverflow=on  OutDataTypeStr=Inherit: Same as input  ParamDataTypeStr=Inherit: Same as input
  Out1 : Outport  VectorParamsAs1DForOutWhenUnconnected=off
  wires:
  In1/1 -> Gain/1
  Gain/1 -> Out1/1

== system ASM_Traffic_new/Environment/Interface_In/ModelSignals/Pos_CP_R2L2_Trailer_CoorSys_E[x;y][m]_ ==
  In1 : Inport
  Gain : Gain  SaturateOnIntegerOverflow=on  OutDataTypeStr=Inherit: Same as input  ParamDataTypeStr=Inherit: Same as input
  Out1 : Outport  VectorParamsAs1DForOutWhenUnconnected=off
  wires:
  Gain/1 -> Out1/1
  In1/1 -> Gain/1

== system ASM_Traffic_new/Environment/Interface_In/ModelSignals/Pos_CP_R2L_CoorSys_E[x;y][m]_ ==
  In1 : Inport
  Gain : Gain  SaturateOnIntegerOverflow=on  OutDataTypeStr=Inherit: Same as input  ParamDataTypeStr=Inherit: Same as input
  Out1 : Outport  VectorParamsAs1DForOutWhenUnconnected=off
  wires:
  Gain/1 -> Out1/1
  In1/1 -> Gain/1

== system ASM_Traffic_new/Environment/Interface_In/ModelSignals/Pos_CP_R2L_Trailer_CoorSys_E[x;y][m]_ ==
  In1 : Inport
  Gain : Gain  SaturateOnIntegerOverflow=on  OutDataTypeStr=Inherit: Same as input  ParamDataTypeStr=Inherit: Same as input
  Out1 : Outport  VectorParamsAs1DForOutWhenUnconnected=off
  wires:
  Gain/1 -> Out1/1
  In1/1 -> Gain/1

== system ASM_Traffic_new/Environment/Interface_In/ModelSignals/Pos_CP_R2R2_CoorSys_E[x;y][m]_ ==
  In1 : Inport
  Gain : Gain  SaturateOnIntegerOverflow=on  OutDataTypeStr=Inherit: Same as input  ParamDataTypeStr=Inherit: Same as input
  Out1 : Outport  VectorParamsAs1DForOutWhenUnconnected=off
  wires:
  In1/1 -> Gain/1
  Gain/1 -> Out1/1

== system ASM_Traffic_new/Environment/Interface_In/ModelSignals/Pos_CP_R2R2_Trailer_CoorSys_E[x;y][m]_ ==
  In1 : Inport
  Gain : Gain  SaturateOnIntegerOverflow=on  OutDataTypeStr=Inherit: Same as input  ParamDataTypeStr=Inherit: Same as input
  Out1 : Outport  VectorParamsAs1DForOutWhenUnconnected=off
  wires:
  Gain/1 -> Out1/1
  In1/1 -> Gain/1

== system ASM_Traffic_new/Environment/Interface_In/ModelSignals/Pos_CP_R2R_CoorSys_E[x;y][m]_ ==
  In1 : Inport
  Gain : Gain  SaturateOnIntegerOverflow=on  OutDataTypeStr=Inherit: Same as input  ParamDataTypeStr=Inherit: Same as input
  Out1 : Outport  VectorParamsAs1DForOutWhenUnconnected=off
  wires:
  Gain/1 -> Out1/1
  In1/1 -> Gain/1

== system ASM_Traffic_new/Environment/Interface_In/ModelSignals/Pos_CP_R2R_Trailer_CoorSys_E[x;y][m]_ ==
  In1 : Inport
  Gain : Gain  SaturateOnIntegerOverflow=on  OutDataTypeStr=Inherit: Same as input  ParamDataTypeStr=Inherit: Same as input
  Out1 : Outport  VectorParamsAs1DForOutWhenUnconnected=off
  wires:
  Gain/1 -> Out1/1
  In1/1 -> Gain/1

== system ASM_Traffic_new/Environment/Interface_In/ModelSignals/Pos_CP_RL2_CoorSys_E[x;y][m]_ ==
  In1 : Inport
  Gain : Gain  SaturateOnIntegerOverflow=on  OutDataTypeStr=Inherit: Same as input  ParamDataTypeStr=Inherit: Same as input
  Out1 : Outport  VectorParamsAs1DForOutWhenUnconnected=off
  wires:
  In1/1 -> Gain/1
  Gain/1 -> Out1/1

== system ASM_Traffic_new/Environment/Interface_In/ModelSignals/Pos_CP_RL2_Trailer_CoorSys_E[x;y][m]_ ==
  In1 : Inport
  Gain : Gain  SaturateOnIntegerOverflow=on  OutDataTypeStr=Inherit: Same as input  ParamDataTypeStr=Inherit: Same as input
  Out1 : Outport  VectorParamsAs1DForOutWhenUnconnected=off
  wires:
  Gain/1 -> Out1/1
  In1/1 -> Gain/1

== system ASM_Traffic_new/Environment/Interface_In/ModelSignals/Pos_CP_RL_CoorSys_E[x;y][m]_ ==
  In1 : Inport
  Gain : Gain  SaturateOnIntegerOverflow=on  OutDataTypeStr=Inherit: Same as input  ParamDataTypeStr=Inherit: Same as input
  Out1 : Outport  VectorParamsAs1DForOutWhenUnconnected=off
  wires:
  Gain/1 -> Out1/1
  In1/1 -> Gain/1

== system ASM_Traffic_new/Environment/Interface_In/ModelSignals/Pos_CP_RL_Trailer_CoorSys_E[x;y][m]_ ==
  In1 : Inport
  Gain : Gain  SaturateOnIntegerOverflow=on  OutDataTypeStr=Inherit: Same as input  ParamDataTypeStr=Inherit: Same as input
  Out1 : Outport  VectorParamsAs1DForOutWhenUnconnected=off
  wires:
  Gain/1 -> Out1/1
  In1/1 -> Gain/1

== system ASM_Traffic_new/Environment/Interface_In/ModelSignals/Pos_CP_RR2_CoorSys_E[x;y][m]_ ==
  In1 : Inport
  Gain : Gain  SaturateOnIntegerOverflow=on  OutDataTypeStr=Inherit: Same as input  ParamDataTypeStr=Inherit: Same as input
  Out1 : Outport  VectorParamsAs1DForOutWhenUnconnected=off
  wires:
  In1/1 -> Gain/1
  Gain/1 -> Out1/1

== system ASM_Traffic_new/Environment/Interface_In/ModelSignals/Pos_CP_RR2_Trailer_CoorSys_E[x;y][m]_ ==
  In1 : Inport
  Gain : Gain  SaturateOnIntegerOverflow=on  OutDataTypeStr=Inherit: Same as input  ParamDataTypeStr=Inherit: Same as input
  Out1 : Outport  VectorParamsAs1DForOutWhenUnconnected=off
  wires:
  Gain/1 -> Out1/1
  In1/1 -> Gain/1

== system ASM_Traffic_new/Environment/Interface_In/ModelSignals/Pos_CP_RR_CoorSys_E[x;y][m]_ ==
  In1 : Inport
  Gain : Gain  SaturateOnIntegerOverflow=on  OutDataTypeStr=Inherit: Same as input  ParamDataTypeStr=Inherit: Same as input
  Out1 : Outport  VectorParamsAs1DForOutWhenUnconnected=off
  wires:
  Gain/1 -> Out1/1
  In1/1 -> Gain/1

== system ASM_Traffic_new/Environment/Interface_In/ModelSignals/Pos_CP_RR_Trailer_CoorSys_E[x;y][m]_ ==
  In1 : Inport
  Gain : Gain  SaturateOnIntegerOverflow=on  OutDataTypeStr=Inherit: Same as input  ParamDataTypeStr=Inherit: Same as input
  Out1 : Outport  VectorParamsAs1DForOutWhenUnconnected=off
  wires:
  Gain/1 -> Out1/1
  In1/1 -> Gain/1

== system ASM_Traffic_new/Environment/Interface_In/ModelSignals/Pos_CP_Rear_CoorSys_E[x;y][m]_ ==
  In1 : Inport
  Gain : Gain  SaturateOnIntegerOverflow=on  OutDataTypeStr=Inherit: Same as input  ParamDataTypeStr=Inherit: Same as input
  Out1 : Outport  VectorParamsAs1DForOutWhenUnconnected=off
  wires:
  Gain/1 -> Out1/1
  In1/1 -> Gain/1

== system ASM_Traffic_new/Environment/Interface_In/ModelSignals/Pos_ClutchPedal[%]_ ==
  In1 : Inport
  DummyGain : Gain  SaturateOnIntegerOverflow=on  OutDataTypeStr=Inherit: Same as input  ParamDataTypeStr=Inherit: Same as input
  Out1 : Outport  VectorParamsAs1DForOutWhenUnconnected=off
  wires:
  In1/1 -> DummyGain/1
  DummyGain/1 -> Out1/1

== system ASM_Traffic_new/Environment/Interface_In/ModelSignals/Pos_Vehicle_CoorSys_E[x;y;z][m]_ ==
  In1 : Inport
  Gain : Gain  SaturateOnIntegerOverflow=on  OutDataTypeStr=Inherit: Same as input  ParamDataTypeStr=Inherit: Same as input
  Out1 : Outport  VectorParamsAs1DForOutWhenUnconnected=off
  wires:
  Gain/1 -> Out1/1
  In1/1 -> Gain/1

== system ASM_Traffic_new/Environment/Interface_In/ModelSignals/RollRate_Vehicle_CoG[deg|s]_ ==
  In1 : Inport
  Gain : Gain  SaturateOnIntegerOverflow=on  OutDataTypeStr=Inherit: Same as input  ParamDataTypeStr=Inherit: Same as input
  Out1 : Outport  VectorParamsAs1DForOutWhenUnconnected=off
  wires:
  Gain/1 -> Out1/1
  In1/1 -> Gain/1

== system ASM_Traffic_new/Environment/Interface_In/ModelSignals/RotationMatrix_V_to_E[1x9]_ ==
  In1 : Inport
  Gain : Gain  SaturateOnIntegerOverflow=on  OutDataTypeStr=Inherit: Same as input  ParamDataTypeStr=Inherit: Same as input
  Out1 : Outport  VectorParamsAs1DForOutWhenUnconnected=off
  wires:
  Gain/1 -> Out1/1
  In1/1 -> Gain/1

== system ASM_Traffic_new/Environment/Interface_In/ModelSignals/SelectorLever[-3T|-2P|-1R|0N|1D]_ ==
  In1 : Inport
  DummyGain : Gain  SaturateOnIntegerOverflow=on  OutDataTypeStr=Inherit: Same as input  ParamDataTypeStr=Inherit: Same as input
  Out1 : Outport  VectorParamsAs1DForOutWhenUnconnected=off
  wires:
  In1/1 -> DummyGain/1
  DummyGain/1 -> Out1/1

== system ASM_Traffic_new/Environment/Interface_In/ModelSignals/Slip_x_Wheel[]_ ==
  In1 : Inport
  DummyGain : Gain  SaturateOnIntegerOverflow=on  OutDataTypeStr=Inherit: Same as input  ParamDataTypeStr=Inherit: Same as input
  Out1 : Outport  VectorParamsAs1DForOutWhenUnconnected=off
  wires:
  In1/1 -> DummyGain/1
  DummyGain/1 -> Out1/1

== system ASM_Traffic_new/Environment/Interface_In/ModelSignals/State_StartButton[-2|-1|0|1|2|3]_ ==
  In1 : Inport
  DummyGain : Gain  SaturateOnIntegerOverflow=on  OutDataTypeStr=Inherit: Same as input  ParamDataTypeStr=Inherit: Same as input
  Out1 : Outport  VectorParamsAs1DForOutWhenUnconnected=off
  wires:
  DummyGain/1 -> Out1/1
  In1/1 -> DummyGain/1

== system ASM_Traffic_new/Environment/Interface_In/ModelSignals/Sw_MasterBrakeCylinder_Mode[1linear|2physical|3Booster]_ ==
  In1 : Inport
  Gain : Gain  SaturateOnIntegerOverflow=on  OutDataTypeStr=Inherit: Same as input  ParamDataTypeStr=Inherit: Same as input
  Out1 : Outport  VectorParamsAs1DForOutWhenUnconnected=off
  wires:
  In1/1 -> Gain/1
  Gain/1 -> Out1/1

== system ASM_Traffic_new/Environment/Interface_In/ModelSignals/Sw_ModelDeskPlottingInterface[0Disabled|1Enabled]_ ==
  In1 : Inport
  Gain : Gain
  Out1 : Outport
  wires:
  Gain/1 -> Out1/1
  In1/1 -> Gain/1

== system ASM_Traffic_new/Environment/Interface_In/ModelSignals/Sw_ModelPortBlocks[0Disabled|1Enabled]_ ==
  In1 : Inport
  Gain : Gain
  Out1 : Outport
  wires:
  Gain/1 -> Out1/1
  In1/1 -> Gain/1

== system ASM_Traffic_new/Environment/Interface_In/ModelSignals/Trq_Engine_1[Nm]_ ==
  In1 : Inport
  DummyGain : Gain  SaturateOnIntegerOverflow=on  OutDataTypeStr=Inherit: Same as input  ParamDataTypeStr=Inherit: Same as input
  Out1 : Outport  VectorParamsAs1DForOutWhenUnconnected=off
  wires:
  DummyGain/1 -> Out1/1
  In1/1 -> DummyGain/1

== system ASM_Traffic_new/Environment/Interface_In/ModelSignals/Trq_Engine_2[Nm]_ ==
  In1 : Inport
  DummyGain : Gain  SaturateOnIntegerOverflow=on  OutDataTypeStr=Inherit: Same as input  ParamDataTypeStr=Inherit: Same as input
  Out1 : Outport  VectorParamsAs1DForOutWhenUnconnected=off
  wires:
  DummyGain/1 -> Out1/1
  In1/1 -> DummyGain/1

== system ASM_Traffic_new/Environment/Interface_In/ModelSignals/Trq_SteeringWheel_SteeringSystem[Nm]_ ==
  In1 : Inport
  Gain : Gain  SaturateOnIntegerOverflow=on  OutDataTypeStr=Inherit: Same as input  ParamDataTypeStr=Inherit: Same as input
  Out1 : Outport  VectorParamsAs1DForOutWhenUnconnected=off
  wires:
  Gain/1 -> Out1/1
  In1/1 -> Gain/1

== system ASM_Traffic_new/Environment/Interface_In/ModelSignals/Type_Engine_1[0Unkown|1Other|2Otto|3Diesel|4Electric]_ ==
  In1 : Inport
  DummyGain : Gain  SaturateOnIntegerOverflow=on  OutDataTypeStr=Inherit: Same as input  ParamDataTypeStr=Inherit: Same as input
  Out1 : Outport  VectorParamsAs1DForOutWhenUnconnected=off
  wires:
  DummyGain/1 -> Out1/1
  In1/1 -> DummyGain/1

== system ASM_Traffic_new/Environment/Interface_In/ModelSignals/Type_Engine_2[0Unkown|1Other|2Otto|3Diesel|4Electric]_ ==
  In1 : Inport
  DummyGain : Gain  SaturateOnIntegerOverflow=on  OutDataTypeStr=Inherit: Same as input  ParamDataTypeStr=Inherit: Same as input
  Out1 : Outport  VectorParamsAs1DForOutWhenUnconnected=off
  wires:
  In1/1 -> DummyGain/1
  DummyGain/1 -> Out1/1

== system ASM_Traffic_new/Environment/Interface_In/ModelSignals/YawRate_Vehicle_CoG[deg|s]_ ==
  In1 : Inport
  Gain : Gain  SaturateOnIntegerOverflow=on  OutDataTypeStr=Inherit: Same as input  ParamDataTypeStr=Inherit: Same as input
  Out1 : Outport  VectorParamsAs1DForOutWhenUnconnected=off
  wires:
  Gain/1 -> Out1/1
  In1/1 -> Gain/1

== system ASM_Traffic_new/Environment/Interface_In/ModelSignals/a_y_Vehicle_CoG[m|s2]_ ==
  In1 : Inport
  Gain : Gain  SaturateOnIntegerOverflow=on  OutDataTypeStr=Inherit: Same as input  ParamDataTypeStr=Inherit: Same as input
  Out1 : Outport  VectorParamsAs1DForOutWhenUnconnected=off
  wires:
  Gain/1 -> Out1/1
  In1/1 -> Gain/1

== system ASM_Traffic_new/Environment/Interface_In/ModelSignals/m_TotalVehicle[kg]_ ==
  In1 : Inport
  DummyGain : Gain  SaturateOnIntegerOverflow=on  OutDataTypeStr=Inherit: Same as input  ParamDataTypeStr=Inherit: Same as input
  Out1 : Outport  VectorParamsAs1DForOutWhenUnconnected=off
  wires:
  DummyGain/1 -> Out1/1
  In1/1 -> DummyGain/1

== system ASM_Traffic_new/Environment/Interface_In/ModelSignals/n_Engine_1[rpm]_ ==
  In1 : Inport
  DummyGain : Gain  SaturateOnIntegerOverflow=on  OutDataTypeStr=Inherit: Same as input  ParamDataTypeStr=Inherit: Same as input
  Out1 : Outport  VectorParamsAs1DForOutWhenUnconnected=off
  wires:
  DummyGain/1 -> Out1/1
  In1/1 -> DummyGain/1

== system ASM_Traffic_new/Environment/Interface_In/ModelSignals/n_Engine_2[rpm]_ ==
  In1 : Inport
  DummyGain : Gain  SaturateOnIntegerOverflow=on  OutDataTypeStr=Inherit: Same as input  ParamDataTypeStr=Inherit: Same as input
  Out1 : Outport  VectorParamsAs1DForOutWhenUnconnected=off
  wires:
  DummyGain/1 -> Out1/1
  In1/1 -> DummyGain/1

== system ASM_Traffic_new/Environment/Interface_In/ModelSignals/omega_Wheel[rad|s]_ ==
  In1 : Inport
  DummyGain : Gain  SaturateOnIntegerOverflow=on  OutDataTypeStr=Inherit: Same as input  ParamDataTypeStr=Inherit: Same as input
  Out1 : Outport  VectorParamsAs1DForOutWhenUnconnected=off
  wires:
  In1/1 -> DummyGain/1
  DummyGain/1 -> Out1/1

== system ASM_Traffic_new/Environment/Interface_In/ModelSignals/r_Dyn_Tire[FL;FR;RL;RR][m]_ ==
  In1 : Inport
  Gain : Gain  SaturateOnIntegerOverflow=on  OutDataTypeStr=Inherit: Same as input  ParamDataTypeStr=Inherit: Same as input
  Out1 : Outport  VectorParamsAs1DForOutWhenUnconnected=off
  wires:
  Gain/1 -> Out1/1
  In1/1 -> Gain/1

== system ASM_Traffic_new/Environment/Interface_In/ModelSignals/s_Preview[m]_ ==
  In1 : Inport
  DummyGain : Gain  SaturateOnIntegerOverflow=on  OutDataTypeStr=Inherit: Same as input  ParamDataTypeStr=Inherit: Same as input
  Out1 : Outport  VectorParamsAs1DForOutWhenUnconnected=off
  wires:
  DummyGain/1 -> Out1/1
  In1/1 -> DummyGain/1

== system ASM_Traffic_new/Environment/Interface_In/ModelSignals/s_Vehicle[m]_ ==
  In1 : Inport
  Gain : Gain  SaturateOnIntegerOverflow=on  OutDataTypeStr=Inherit: Same as input  ParamDataTypeStr=Inherit: Same as input
  Out1 : Outport  VectorParamsAs1DForOutWhenUnconnected=off
  wires:
  Gain/1 -> Out1/1
  In1/1 -> Gain/1

== system ASM_Traffic_new/Environment/Interface_In/ModelSignals/t_Preview_vRef_Driver[s]_ ==
  In1 : Inport
  DummyGain : Gain  SaturateOnIntegerOverflow=on  OutDataTypeStr=Inherit: Same as input  ParamDataTypeStr=Inherit: Same as input
  Out1 : Outport  VectorParamsAs1DForOutWhenUnconnected=off
  wires:
  DummyGain/1 -> Out1/1
  In1/1 -> DummyGain/1

== system ASM_Traffic_new/Environment/Interface_In/ModelSignals/v_x_Vehicle_CoG[km|h]_ ==
  In1 : Inport
  Gain : Gain  SaturateOnIntegerOverflow=on  OutDataTypeStr=Inherit: Same as input  ParamDataTypeStr=Inherit: Same as input
  Out1 : Outport  VectorParamsAs1DForOutWhenUnconnected=off
  wires:
  Gain/1 -> Out1/1
  In1/1 -> Gain/1

== system ASM_Traffic_new/Environment/Interface_In/ModelSignals/v_y_Vehicle_CoG[km|h]_ ==
  In1 : Inport
  Gain : Gain  SaturateOnIntegerOverflow=on  OutDataTypeStr=Inherit: Same as input  ParamDataTypeStr=Inherit: Same as input
  Out1 : Outport  VectorParamsAs1DForOutWhenUnconnected=off
  wires:
  Gain/1 -> Out1/1
  In1/1 -> Gain/1

== system ASM_Traffic_new/Environment/Interface_Out/Animation/ASM_Vehicle_TurnLights[]_ ==
  In1 : Inport
  Gain : Gain  SaturateOnIntegerOverflow=on  OutDataTypeStr=Inherit: Same as input  ParamDataTypeStr=Inherit: Same as input
  Out1 : Outport  VectorParamsAs1DForOutWhenUnconnected=off
  wires:
  Gain/1 -> Out1/1
  In1/1 -> Gain/1

== system ASM_Traffic_new/Environment/Interface_Out/Animation/Distance_MeasPnt_Marker_Left[m]_ ==
  In1 : Inport
  Gain : Gain  SaturateOnIntegerOverflow=on  OutDataTypeStr=Inherit: Same as input  ParamDataTypeStr=Inherit: Same as input
  Out1 : Outport  VectorParamsAs1DForOutWhenUnconnected=off
  wires:
  In1/1 -> Gain/1
  Gain/1 -> Out1/1

== system ASM_Traffic_new/Environment/Interface_Out/Animation/Distance_MeasPnt_Marker_Right[m]_ ==
  In1 : Inport
  Gain : Gain  SaturateOnIntegerOverflow=on  OutDataTypeStr=Inherit: Same as input  ParamDataTypeStr=Inherit: Same as input
  Out1 : Outport  VectorParamsAs1DForOutWhenUnconnected=off
  wires:
  Gain/1 -> Out1/1
  In1/1 -> Gain/1

== system ASM_Traffic_new/Environment/Interface_Out/Animation/Flag_FellowUsed[0|1]_ ==
  In1 : Inport
  Gain : Gain  SaturateOnIntegerOverflow=on  OutDataTypeStr=Inherit: Same as input  ParamDataTypeStr=Inherit: Same as input
  Out1 : Outport  VectorParamsAs1DForOutWhenUnconnected=off
  wires:
  In1/1 -> Gain/1
  Gain/1 -> Out1/1

== system ASM_Traffic_new/Environment/Interface_Out/Animation/ManeuverState[]_ ==
  In1 : Inport
  Gain : Gain  SaturateOnIntegerOverflow=on  OutDataTypeStr=Inherit: Same as input  ParamDataTypeStr=Inherit: Same as input
  Out1 : Outport  VectorParamsAs1DForOutWhenUnconnected=off
  wires:
  Gain/1 -> Out1/1
  In1/1 -> Gain/1

== system ASM_Traffic_new/Environment/Interface_Out/Animation/ManeuverTime[s]_ ==
  In1 : Inport
  Gain : Gain  SaturateOnIntegerOverflow=on  OutDataTypeStr=Inherit: Same as input  ParamDataTypeStr=Inherit: Same as input
  Out1 : Outport  VectorParamsAs1DForOutWhenUnconnected=off
  wires:
  In1/1 -> Gain/1
  Gain/1 -> Out1/1

== system ASM_Traffic_new/Environment/Interface_Out/Animation/MarkerType_Left[]_ ==
  In1 : Inport
  Gain : Gain  SaturateOnIntegerOverflow=on  OutDataTypeStr=Inherit: Same as input  ParamDataTypeStr=Inherit: Same as input
  Out1 : Outport  VectorParamsAs1DForOutWhenUnconnected=off
  wires:
  Gain/1 -> Out1/1
  In1/1 -> Gain/1

== system ASM_Traffic_new/Environment/Interface_Out/Animation/MarkerType_Right[]_ ==
  In1 : Inport
  Gain : Gain  SaturateOnIntegerOverflow=on  OutDataTypeStr=Inherit: Same as input  ParamDataTypeStr=Inherit: Same as input
  Out1 : Outport  VectorParamsAs1DForOutWhenUnconnected=off
  wires:
  In1/1 -> Gain/1
  Gain/1 -> Out1/1

== system ASM_Traffic_new/Environment/Interface_Out/Animation/Mnv_DoorFL[]_ ==
  In1 : Inport
  Gain : Gain  SaturateOnIntegerOverflow=on  OutDataTypeStr=Inherit: Same as input  ParamDataTypeStr=Inherit: Same as input
  Out1 : Outport  VectorParamsAs1DForOutWhenUnconnected=off
  wires:
  Gain/1 -> Out1/1
  In1/1 -> Gain/1

== system ASM_Traffic_new/Environment/Interface_Out/Animation/Mnv_DoorFR[]_ ==
  In1 : Inport
  Gain : Gain  SaturateOnIntegerOverflow=on  OutDataTypeStr=Inherit: Same as input  ParamDataTypeStr=Inherit: Same as input
  Out1 : Outport  VectorParamsAs1DForOutWhenUnconnected=off
  wires:
  Gain/1 -> Out1/1
  In1/1 -> Gain/1

== system ASM_Traffic_new/Environment/Interface_Out/Animation/Mnv_DoorRL[]_ ==
  In1 : Inport
  Gain : Gain  SaturateOnIntegerOverflow=on  OutDataTypeStr=Inherit: Same as input  ParamDataTypeStr=Inherit: Same as input
  Out1 : Outport  VectorParamsAs1DForOutWhenUnconnected=off
  wires:
  Gain/1 -> Out1/1
  In1/1 -> Gain/1

== system ASM_Traffic_new/Environment/Interface_Out/Animation/Mnv_DoorRR[]_ ==
  In1 : Inport
  Gain : Gain  SaturateOnIntegerOverflow=on  OutDataTypeStr=Inherit: Same as input  ParamDataTypeStr=Inherit: Same as input
  Out1 : Outport  VectorParamsAs1DForOutWhenUnconnected=off
  wires:
  Gain/1 -> Out1/1
  In1/1 -> Gain/1

== system ASM_Traffic_new/Environment/Interface_Out/Animation/Mnv_Hood[]_ ==
  In1 : Inport
  Gain : Gain  SaturateOnIntegerOverflow=on  OutDataTypeStr=Inherit: Same as input  ParamDataTypeStr=Inherit: Same as input
  Out1 : Outport  VectorParamsAs1DForOutWhenUnconnected=off
  wires:
  In1/1 -> Gain/1
  Gain/1 -> Out1/1
